simulink model "spherical_wrist"  (R2024b)
settings: Solver=ode23t  StartTime=0.0  StopTime=100  FixedStep=0.001  RelTol=1e-3
InitFcn:
  | WRIST_mk2_1_DataFile
model workspace (MAT data in the model file):
  Damp : Simulink.Parameter (value not decoded)
  Dm : Simulink.Parameter (value not decoded)
  Jm : Simulink.Parameter (value not decoded)
  Km : Simulink.Parameter (value not decoded)
  Tc : Simulink.Parameter (value not decoded)
symbols that are objects in the model workspace (value not decoded): Damp, Dm, Tc
undefined symbols (not defined in the file or in its folder): smiData, X, Y, Z
libraries: sm_lib x370, nesl_utility x32, fl_lib x15, sdl_lib x9, simulink_extras x4, sharedtransform x2, slpidlib x1
(part 10 of 10)

== system spherical_wrist/NewWrist21/ROD 3/SPINA ROD 3 ==
  ReferenceFrame : sm_lib/Frames and Transforms/Reference Frame
  Solid : sm_lib/Body Elements/File Solid  ExtGeomFileName=ic_021_p_196_prt.step  UnitType=FromFile  ExtGeomFileUnits=m  StepReaderType=HEX  ExportConvexHullGeometry=off  InertiaType=Custom  BasedOnType=DensityFromFile  Density=1000  DensityUnits=kg/m^3  Mass=smiData.Solid(5).mass  MassUnits=kg  CenterOfMass=smiData.Solid(5).CoM  CenterOfMassUnits=mm  MomentsOfInertia=smiData.Solid(5).MoI  MomentsOfInertiaUnits=kg*mm^2  ProductsOfInertia=smiData.Solid(5).PoI  ProductsOfInertiaUnits=kg*mm^2  GraphicType=FromGeometry  MarkerShape=Sphere  MarkerSize=10  GraphicVisPropType=SimpleVisualProperties  GraphicDiffuseColor=smiData.Solid(5).color  GraphicOpacity=smiData.Solid(5).opacity  GraphicSpecularColor=[0.5 0.5 0.5 1.0]  GraphicAmbientColor=[0.15 0.15 0.15 1.0]  GraphicEmissiveColor=[0.0 0.0 0.0 1.0]  GraphicShininess=75  DoExposeReferenceFrame=on  SerializedFrames=<Frames/>
  Transform : sm_lib/Frames and Transforms/Rigid Transform  RotationMethod=ArbitraryAxis  FollAlignAxisA=+X  BaseAlignAxisA=+Y  FollAlignAxisB=+Y  BaseAlignAxisB=+Z  RotationStandardAxis=+Z  RotationAngle=smiData.RigidTransform(8).angle  RotationAngleUnits=rad  RotationArbitraryAxis=smiData.RigidTransform(8).axis  RotationSequenceAxes=FollowerAxes  RotationSequence=XYX  RotationSequenceAngles=[0 0 0]  RotationSequenceAnglesUnits=deg  RotationMatrix=[1 0 0;0 1 0;0 0 1]  Quaternion=[1 0 0 0]  TranslationMethod=Cartesian  TranslationCartesianOffset=smiData.RigidTransform(8).translation  TranslationCartesianOffsetUnits=mm  TranslationStandardAxis=+Z  TranslationStandardOffset=0  TranslationStandardOffsetUnits=m  TranslationROffset=0  TranslationROffsetUnits=m  TranslationThetaOffset=0  TranslationThetaOffsetUnits=deg  TranslationZOffset=0  TranslationZOffsetUnits=m
  F : PMIOPort  Side=Left
  connections:
  Solid/RConn1 -- ReferenceFrame/RConn1 -- Transform/LConn1
  Transform/RConn1 -- F/RConn1

== system spherical_wrist/NewWrist21/ROD 3/x618_4_RIGID ==
  ReferenceFrame : sm_lib/Frames and Transforms/Reference Frame
  Solid : sm_lib/Body Elements/File Solid  ExtGeomFileName=618-4_prt.step  UnitType=FromFile  ExtGeomFileUnits=m  StepReaderType=HEX  ExportConvexHullGeometry=off  InertiaType=Custom  BasedOnType=DensityFromFile  Density=1000  DensityUnits=kg/m^3  Mass=smiData.Solid(4).mass  MassUnits=kg  CenterOfMass=smiData.Solid(4).CoM  CenterOfMassUnits=mm  MomentsOfInertia=smiData.Solid(4).MoI  MomentsOfInertiaUnits=kg*mm^2  ProductsOfInertia=smiData.Solid(4).PoI  ProductsOfInertiaUnits=kg*mm^2  GraphicType=FromGeometry  MarkerShape=Sphere  MarkerSize=10  GraphicVisPropType=SimpleVisualProperties  GraphicDiffuseColor=smiData.Solid(4).color  GraphicOpacity=smiData.Solid(4).opacity  GraphicSpecularColor=[0.5 0.5 0.5 1.0]  GraphicAmbientColor=[0.15 0.15 0.15 1.0]  GraphicEmissiveColor=[0.0 0.0 0.0 1.0]  GraphicShininess=75  DoExposeReferenceFrame=on  SerializedFrames=<Frames/>
  F : PMIOPort  Side=Left
  connections:
  Solid/RConn1 -- ReferenceFrame/RConn1 -- F/RConn1

== system spherical_wrist/NewWrist21/ROD 3/x618_4_RIGID1 ==
  ReferenceFrame : sm_lib/Frames and Transforms/Reference Frame
  Solid : sm_lib/Body Elements/File Solid  ExtGeomFileName=618-4_prt.step  UnitType=FromFile  ExtGeomFileUnits=m  StepReaderType=HEX  ExportConvexHullGeometry=off  InertiaType=Custom  BasedOnType=DensityFromFile  Density=1000  DensityUnits=kg/m^3  Mass=smiData.Solid(4).mass  MassUnits=kg  CenterOfMass=smiData.Solid(4).CoM  CenterOfMassUnits=mm  MomentsOfInertia=smiData.Solid(4).MoI  MomentsOfInertiaUnits=kg*mm^2  ProductsOfInertia=smiData.Solid(4).PoI  ProductsOfInertiaUnits=kg*mm^2  GraphicType=FromGeometry  MarkerShape=Sphere  MarkerSize=10  GraphicVisPropType=SimpleVisualProperties  GraphicDiffuseColor=smiData.Solid(4).color  GraphicOpacity=smiData.Solid(4).opacity  GraphicSpecularColor=[0.5 0.5 0.5 1.0]  GraphicAmbientColor=[0.15 0.15 0.15 1.0]  GraphicEmissiveColor=[0.0 0.0 0.0 1.0]  GraphicShininess=75  DoExposeReferenceFrame=on  SerializedFrames=<Frames/>
  F : PMIOPort  Side=Left
  connections:
  Solid/RConn1 -- ReferenceFrame/RConn1 -- F/RConn1

== system spherical_wrist/NewWrist21/ROD 3/x618_4_RIGID2 ==
  ReferenceFrame : sm_lib/Frames and Transforms/Reference Frame
  Solid : sm_lib/Body Elements/File Solid  ExtGeomFileName=618-4_prt.step  UnitType=FromFile  ExtGeomFileUnits=m  StepReaderType=HEX  ExportConvexHullGeometry=off  InertiaType=Custom  BasedOnType=DensityFromFile  Density=1000  DensityUnits=kg/m^3  Mass=smiData.Solid(4).mass  MassUnits=kg  CenterOfMass=smiData.Solid(4).CoM  CenterOfMassUnits=mm  MomentsOfInertia=smiData.Solid(4).MoI  MomentsOfInertiaUnits=kg*mm^2  ProductsOfInertia=smiData.Solid(4).PoI  ProductsOfInertiaUnits=kg*mm^2  GraphicType=FromGeometry  MarkerShape=Sphere  MarkerSize=10  GraphicVisPropType=SimpleVisualProperties  GraphicDiffuseColor=smiData.Solid(4).color  GraphicOpacity=smiData.Solid(4).opacity  GraphicSpecularColor=[0.5 0.5 0.5 1.0]  GraphicAmbientColor=[0.15 0.15 0.15 1.0]  GraphicEmissiveColor=[0.0 0.0 0.0 1.0]  GraphicShininess=75  DoExposeReferenceFrame=on  SerializedFrames=<Frames/>
  Transform : sm_lib/Frames and Transforms/Rigid Transform  RotationMethod=ArbitraryAxis  FollAlignAxisA=+X  BaseAlignAxisA=+Y  FollAlignAxisB=+Y  BaseAlignAxisB=+Z  RotationStandardAxis=+Z  RotationAngle=smiData.RigidTransform(34).angle  RotationAngleUnits=rad  RotationArbitraryAxis=smiData.RigidTransform(34).axis  RotationSequenceAxes=FollowerAxes  RotationSequence=XYX  RotationSequenceAngles=[0 0 0]  RotationSequenceAnglesUnits=deg  RotationMatrix=[1 0 0;0 1 0;0 0 1]  Quaternion=[1 0 0 0]  TranslationMethod=Cartesian  TranslationCartesianOffset=smiData.RigidTransform(34).translation  TranslationCartesianOffsetUnits=mm  TranslationStandardAxis=+Z  TranslationStandardOffset=0  TranslationStandardOffsetUnits=m  TranslationROffset=0  TranslationROffsetUnits=m  TranslationThetaOffset=0  TranslationThetaOffsetUnits=deg  TranslationZOffset=0  TranslationZOffsetUnits=m
  Transform1 : sm_lib/Frames and Transforms/Rigid Transform  RotationMethod=ArbitraryAxis  FollAlignAxisA=+X  BaseAlignAxisA=+Y  FollAlignAxisB=+Y  BaseAlignAxisB=+Z  RotationStandardAxis=+Z  RotationAngle=smiData.RigidTransform(51).angle  RotationAngleUnits=rad  RotationArbitraryAxis=smiData.RigidTransform(51).axis  RotationSequenceAxes=FollowerAxes  RotationSequence=XYX  RotationSequenceAngles=[0 0 0]  RotationSequenceAnglesUnits=deg  RotationMatrix=[1 0 0;0 1 0;0 0 1]  Quaternion=[1 0 0 0]  TranslationMethod=Cartesian  TranslationCartesianOffset=smiData.RigidTransform(51).translation  TranslationCartesianOffsetUnits=mm  TranslationStandardAxis=+Z  TranslationStandardOffset=0  TranslationStandardOffsetUnits=m  TranslationROffset=0  TranslationROffsetUnits=m  TranslationThetaOffset=0  TranslationThetaOffsetUnits=deg  TranslationZOffset=0  TranslationZOffsetUnits=m
  F1 : PMIOPort  Side=Left
  F : PMIOPort  Port=2  Side=Left
  connections:
  Solid/RConn1 -- ReferenceFrame/RConn1 -- Transform/LConn1 -- Transform1/LConn1
  Transform/RConn1 -- F/RConn1
  Transform1/RConn1 -- F1/RConn1

== system spherical_wrist/NewWrist21/ROD 3/x618_4_RIGID3 ==
  ReferenceFrame : sm_lib/Frames and Transforms/Reference Frame
  Solid : sm_lib/Body Elements/File Solid  ExtGeomFileName=618-4_prt.step  UnitType=FromFile  ExtGeomFileUnits=m  StepReaderType=HEX  ExportConvexHullGeometry=off  InertiaType=Custom  BasedOnType=DensityFromFile  Density=1000  DensityUnits=kg/m^3  Mass=smiData.Solid(4).mass  MassUnits=kg  CenterOfMass=smiData.Solid(4).CoM  CenterOfMassUnits=mm  MomentsOfInertia=smiData.Solid(4).MoI  MomentsOfInertiaUnits=kg*mm^2  ProductsOfInertia=smiData.Solid(4).PoI  ProductsOfInertiaUnits=kg*mm^2  GraphicType=FromGeometry  MarkerShape=Sphere  MarkerSize=10  GraphicVisPropType=SimpleVisualProperties  GraphicDiffuseColor=smiData.Solid(4).color  GraphicOpacity=smiData.Solid(4).opacity  GraphicSpecularColor=[0.5 0.5 0.5 1.0]  GraphicAmbientColor=[0.15 0.15 0.15 1.0]  GraphicEmissiveColor=[0.0 0.0 0.0 1.0]  GraphicShininess=75  DoExposeReferenceFrame=on  SerializedFrames=<Frames/>
  Transform : sm_lib/Frames and Transforms/Rigid Transform  RotationMethod=ArbitraryAxis  FollAlignAxisA=+X  BaseAlignAxisA=+Y  FollAlignAxisB=+Y  BaseAlignAxisB=+Z  RotationStandardAxis=+Z  RotationAngle=smiData.RigidTransform(46).angle  RotationAngleUnits=rad  RotationArbitraryAxis=smiData.RigidTransform(46).axis  RotationSequenceAxes=FollowerAxes  RotationSequence=XYX  RotationSequenceAngles=[0 0 0]  RotationSequenceAnglesUnits=deg  RotationMatrix=[1 0 0;0 1 0;0 0 1]  Quaternion=[1 0 0 0]  TranslationMethod=Cartesian  TranslationCartesianOffset=smiData.RigidTransform(46).translation  TranslationCartesianOffsetUnits=mm  TranslationStandardAxis=+Z  TranslationStandardOffset=0  TranslationStandardOffsetUnits=m  TranslationROffset=0  TranslationROffsetUnits=m  TranslationThetaOffset=0  TranslationThetaOffsetUnits=deg  TranslationZOffset=0  TranslationZOffsetUnits=m
  Transform1 : sm_lib/Frames and Transforms/Rigid Transform  RotationMethod=ArbitraryAxis  FollAlignAxisA=+X  BaseAlignAxisA=+Y  FollAlignAxisB=+Y  BaseAlignAxisB=+Z  RotationStandardAxis=+Z  RotationAngle=smiData.RigidTransform(57).angle  RotationAngleUnits=rad  RotationArbitraryAxis=smiData.RigidTransform(57).axis  RotationSequenceAxes=FollowerAxes  RotationSequence=XYX  RotationSequenceAngles=[0 0 0]  RotationSequenceAnglesUnits=deg  RotationMatrix=[1 0 0;0 1 0;0 0 1]  Quaternion=[1 0 0 0]  TranslationMethod=Cartesian  TranslationCartesianOffset=smiData.RigidTransform(57).translation  TranslationCartesianOffsetUnits=mm  TranslationStandardAxis=+Z  TranslationStandardOffset=0  TranslationStandardOffsetUnits=m  TranslationROffset=0  TranslationROffsetUnits=m  TranslationThetaOffset=0  TranslationThetaOffsetUnits=deg  TranslationZOffset=0  TranslationZOffsetUnits=m
  F1 : PMIOPort  Side=Left
  F : PMIOPort  Port=2  Side=Left
  connections:
  Solid/RConn1 -- ReferenceFrame/RConn1 -- Transform/LConn1 -- Transform1/LConn1
  Transform/RConn1 -- F/RConn1
  Transform1/RConn1 -- F1/RConn1

== system spherical_wrist/Position_Controller/wrapTo180Simulink/singleWrapTo180_1 ==
  angle : Inport
  Add6 : Sum  Inputs=-+
  Add7 : Sum
  Constant : Constant  Value=360
  Constant4 : Constant  Value=180
  Constant5 : Constant  Value=360
  Constant6 : Constant  Value=-180
  Relational Operator : RelationalOperator  Operator=>  OutDataTypeStr=boolean  RndMeth=Simplest  InputSameDT=off
  Relational Operator1 : RelationalOperator  Operator=<  OutDataTypeStr=boolean  RndMeth=Simplest  InputSameDT=off
  Switch4 : Switch  Criteria=u2 > Threshold  SaturateOnIntegerOverflow=off  InputSameDT=off
  Switch5 : Switch  Criteria=u2 > Threshold  SaturateOnIntegerOverflow=off  InputSameDT=off
  wrappedAngle : Outport
  wires:
  Relational Operator/1 -> Switch4/2
  Constant5/1 -> Add6/1
  Switch5/1 -> wrappedAngle/1
  Add7/1 -> Switch5/1
  Constant4/1 -> Relational Operator/2
  Switch4/1 -> Switch5/3
  Constant/1 -> Add7/2
  Add6/1 -> Switch4/1
  angle/1 -> Switch4/3, Relational Operator/1, Add6/2, Add7/1, Relational Operator1/1
  Constant6/1 -> Relational Operator1/2
  Relational Operator1/1 -> Switch5/2

== system spherical_wrist/Position_Controller/wrapTo180Simulink/singleWrapTo180_2 ==
  angle : Inport
  Add6 : Sum  Inputs=-+
  Add7 : Sum
  Constant : Constant  Value=360
  Constant4 : Constant  Value=180
  Constant5 : Constant  Value=360
  Constant6 : Constant  Value=-180
  Relational Operator : RelationalOperator  Operator=>  OutDataTypeStr=boolean  RndMeth=Simplest  InputSameDT=off
  Relational Operator1 : RelationalOperator  Operator=<  OutDataTypeStr=boolean  RndMeth=Simplest  InputSameDT=off
  Switch4 : Switch  Criteria=u2 > Threshold  SaturateOnIntegerOverflow=off  InputSameDT=off
  Switch5 : Switch  Criteria=u2 > Threshold  SaturateOnIntegerOverflow=off  InputSameDT=off
  wrappedAngle : Outport
  wires:
  Relational Operator/1 -> Switch4/2
  Constant5/1 -> Add6/1
  Switch5/1 -> wrappedAngle/1
  Add7/1 -> Switch5/1
  Constant4/1 -> Relational Operator/2
  Switch4/1 -> Switch5/3
  Constant/1 -> Add7/2
  Add6/1 -> Switch4/1
  angle/1 -> Switch4/3, Relational Operator/1, Add6/2, Add7/1, Relational Operator1/1
  Constant6/1 -> Relational Operator1/2
  Relational Operator1/1 -> Switch5/2

== system spherical_wrist/Position_Controller/wrapTo180Simulink/singleWrapTo180_3 ==
  angle : Inport
  Add6 : Sum  Inputs=-+
  Add7 : Sum
  Constant : Constant  Value=360
  Constant4 : Constant  Value=180
  Constant5 : Constant  Value=360
  Constant6 : Constant  Value=-180
  Relational Operator : RelationalOperator  Operator=>  OutDataTypeStr=boolean  RndMeth=Simplest  InputSameDT=off
  Relational Operator1 : RelationalOperator  Operator=<  OutDataTypeStr=boolean  RndMeth=Simplest  InputSameDT=off
  Switch4 : Switch  Criteria=u2 > Threshold  SaturateOnIntegerOverflow=off  InputSameDT=off
  Switch5 : Switch  Criteria=u2 > Threshold  SaturateOnIntegerOverflow=off  InputSameDT=off
  wrappedAngle : Outport
  wires:
  Relational Operator/1 -> Switch4/2
  Constant5/1 -> Add6/1
  Switch5/1 -> wrappedAngle/1
  Add7/1 -> Switch5/1
  Constant4/1 -> Relational Operator/2
  Switch4/1 -> Switch5/3
  Constant/1 -> Add7/2
  Add6/1 -> Switch4/1
  angle/1 -> Switch4/3, Relational Operator/1, Add6/2, Add7/1, Relational Operator1/1
  Constant6/1 -> Relational Operator1/2
  Relational Operator1/1 -> Switch5/2

== matlab function spherical_wrist/Position_Controller/wrapTo180 ==
  data: u input; y output
function y = wrap(u)

y = u;

for i=1:3
    while y(i) > 180.0
        y(i) = y(i) - 360.0;
    end

    while y(i) < -180.0
        y(i) = y(i) + 360.0;
    end
end

== matlab function spherical_wrist/Position_Controller/wrist_decoupler/ypr2motors ==
  data: ypr input; theta output; out_of_range output; theta_off input; plat_off input; arm_bend input
function [theta,out_of_range] = ypr2motors(ypr, theta_off, plat_off, arm_bend)

persistent Pz;
persistent PQ;
persistent Q;
persistent last_theta_ok;

if isempty(Pz)
    Pz = -tand(arm_bend)*[1; 1; 1];
    P = [cosd(theta_off) sind(theta_off) Pz];
    Q = [cosd(plat_off) sind(plat_off) [0; 0; 0]];
    PQ = [P(1,:)*Q(1,:)' P(2,:)*Q(2,:)' P(3,:)*Q(3,:)'];
    last_theta_ok = [0;0;0];
end

q = Q*eul2rotm(deg2rad(ypr'))';

m = [sqrt(q(1,1)^2+q(1,2)^2) sqrt(q(2,1)^2+q(2,2)^2) sqrt(q(3,1)^2+q(3,2)^2)];

if min(abs(m)) == 0
    % out of mechanical motion range
    theta = last_theta_ok;
    out_of_range = 1;
    return;
end

arg = [(PQ(1)-Pz(1)*q(1,3))/m(1); (PQ(2)-Pz(2)*q(2,3))/m(2); (PQ(3)-Pz(3)*q(3,3))/m(3)];

if max(abs(arg)) > 0.99
    % out of mechanical motion range
    theta = last_theta_ok;
    out_of_range = 2;
    return;
end

theta = atan2d(q(:,2),q(:,1))+[90; 90; 90;]-asind(arg);

gap = abs(Wrap180([(theta(2)-theta(1)) (theta(3)-theta(2)) (theta(1)-theta(3))]));

if min(gap) < 33.0
    % out of mechanical motion range
    theta = last_theta_ok;
    out_of_range = 3;
    return;
end

theta = Wrap180(theta-theta_off);

last_theta_ok = theta;
        
out_of_range = 0;

end

%%%%%%%%%%%%%%%%%%%%%%%

function y = Wrap180(x)

    y = x;

    for i=1:3
        while y(i) > 180.0
            y(i) = y(i) - 360.0;
        end
 
        while y(i) < -180.0
            y(i) = y(i) + 360.0;
        end
    end
end

== matlab function spherical_wrist/Position_Controller/wrist_decoupler/motors2ypr ==
  settings: sampleTime=0.1
  data: theta_diff input; theta_off input; attitude output; singularity output; cycles output; plat_off input; arm_bend input
function [attitude,singularity,cycles] = motors2ypr(theta_diff, theta_off, plat_off, arm_bend)

persistent Q;
persistent PQ;
persistent Pz;
persistent T;
persistent attitude_ok;

theta_diff = Wrap180(theta_diff);

if isempty(Q)
    Pz = -tand(arm_bend)*[1; 1; 1];
    P = [cosd(theta_off) sind(theta_off) Pz];
    Q = [cosd(plat_off) sind(plat_off) [0; 0; 0]];
    PQ = [P(1,:)*Q(1,:)' P(2,:)*Q(2,:)' P(3,:)*Q(3,:)'];

    hyaw = 0.1666*(theta_diff(1)+theta_diff(2)+theta_diff(3));
    T = quaternion(cosd(hyaw),0,0,sind(0.5*hyaw));
    attitude_ok = compact(T);
end

%%%%%%%%%%%%%%%%%%%%%%%%%%%%%%%%%%%%%%%%%%%%%%%%%%%%

%%%%%%%%%%%%%%%%%%%%%%%%%%%%%%%%%%%%%%%%%%%%%%%%%%%%

%hyaw = 0.1666*(theta_diff(1)+theta_diff(2)+theta_diff(3));
%T = quaternion(cosd(hyaw),0,0,sind(0.5*hyaw));
%T = quaternion(1,0,0,0);

Told = T;

singularity = 0;

step = 0.01;

first_try = true;

for cycles=1:40
    
    q = rotatepoint(T,Q);
    
    %%%%%%%%%%%%%%%%%%%%%%%%%%%%%%%%%%%%%%%%%%%%%%%%%%%%%%%%%%%%%%%%%%%%%%%
    
    m = [sqrt(q(1,1)^2+q(1,2)^2) sqrt(q(2,1)^2+q(2,2)^2) sqrt(q(3,1)^2+q(3,2)^2)];

    if min(abs(m)) == 0
        % out of mechanical motion range
        if step > 0.001
            step = 0.5*step;
            T = Told;
            continue;
        elseif first_try
            first_try = false;
            step = 0.01;
            hyaw = 0.1666*(theta_diff(1)+theta_diff(2)+theta_diff(3));
            T = quaternion(cosd(hyaw),0,0,sind(0.5*hyaw));
            continue;
        end
        
        break;
    end
    
    arg = [(PQ(1)-Pz(1)*q(1,3))/m(1); (PQ(2)-Pz(2)*q(2,3))/m(2); (PQ(3)-Pz(3)*q(3,3))/m(3)];
    
    if max(abs(arg)) > 1.0
        % out of mechanical motion range
        if step > 0.001
            step = 0.5*step;
            T = Told;
            continue;
        elseif first_try
            first_try = false;
            step = 0.01;
            hyaw = 0.1666*(theta_diff(1)+theta_diff(2)+theta_diff(3));
            T = quaternion(cosd(hyaw),0,0,sind(0.5*hyaw));
            continue;
        end

        break;
    end
    
    theta = atan2d(q(:,2),q(:,1))+[90; 90; 90;]-asind(arg);
    
    %%%%%%%%%%%%%%%%%%%%%%%%%%%%%%%%%%%%%%%%%%%%%%%%%%%%%%%%%%%%%%%%%%%%%%%
    
    theta_err = Wrap180(theta_diff+theta_off-theta);
       
    if max(abs(theta_err)) < 0.1
        T = normalize(T);
        attitude = compact(T);
        attitude_ok = attitude;
        return;
    end
        
    p = [cosd(theta) sind(theta) Pz];
        
    q1xp1 = cross(q(1,:),p(1,:));
    q2xp2 = cross(q(2,:),p(2,:));
    q3xp3 = cross(q(3,:),p(3,:));
        
    if min(abs([q1xp1(3) q2xp2(3) q3xp3(3)])) == 0.0
        % ill jacobian
        if step > 0.001
            step = 0.5*step;
            T = Told;
            continue;
        elseif first_try
            first_try = false;
            step = 0.01;
            hyaw = 0.1666*(theta_diff(1)+theta_diff(2)+theta_diff(3));
            T = quaternion(cosd(hyaw),0,0,sind(0.5*hyaw));
            continue;
        end

        break;
    end
        
    if det([q1xp1/q1xp1(3); q2xp2/q2xp2(3); q3xp3/q3xp3(3)]) == 0.0
        % ill jacobian
        if step > 0.001
            step = 0.5*step;
            T = Told;
            continue;
        elseif first_try
            first_try = false;
            step = 0.01;
            hyaw = 0.1666*(theta_diff(1)+theta_diff(2)+theta_diff(3));
            T = quaternion(cosd(hyaw),0,0,sind(0.5*hyaw));
            continue;
        end

        break;
    end
        
    Told = T;
    T = quaternion(([q1xp1/q1xp1(3); q2xp2/q2xp2(3); q3xp3/q3xp3(3)]\(step*theta_err))','rotvec')*T;
end

T = quaternion(1,0,0,0);
attitude = attitude_ok;
singularity = 1;

end

%%%%%%%%%%%%%%%%%%%%%%%

function y = Wrap180(x)

    y = x;

    for i=1:3
        while y(i) >= 180.0
            y(i) = y(i) - 360.0;
        end
 
        while y(i) < -180.0
            y(i) = y(i) + 360.0;
        end
    end
end
